simulink model "BoostPFC_Design_HoldUpTest"  (R2024b)
settings: Solver=FixedStepDiscrete  StartTime=0  StopTime=sim_stop_time  FixedStep=Ts_sim  RelTol=1e-3
InitFcn:
  | modelFile=get_param(bdroot,'FileName'); run(fullfile(fileparts(modelFile),'BoostPFC_Design_HoldUp_Init.m')); clear modelFile
values from neighbouring files (symbols this model uses):
  actual_peak_cycle_limit_A = 4.00    (= 4)    [BoostPFC_Design_ControlledStartup_Init.m]
  actual_peak_fault_limit_A = 4.50    (= 4.5)    [BoostPFC_Design_ControlledStartup_Init.m]
  C_out = 2200e-6    (= 0.0022)    [BoostPFC_Design_Init.m]
  duty_max = 0.95    [BoostPFC_Design_Init.m]
  duty_min = 0.0    (= 0)    [BoostPFC_Design_Init.m]
  f_line = 50    [BoostPFC_Design_Init.m]
  f_sw = 50e3    (= 50000)    [BoostPFC_Design_Init.m]
  hold_up_command_time_s = 1.200    (= 1.2)    [BoostPFC_Design_HoldUp_Init.m]
  Ipk_limit = 4.5    [BoostPFC_Design_Init.m]
  Ki_i = Kp_i*2*pi*fz_i    (= 695.807110277)    [BoostPFC_Design_Init.m]
  Ki_v = Kp_v*2*pi*fz_v    [BoostPFC_Design_Init.m]
  Kp_i = 2*pi*fc_i_target*L_boost/Vout_ref    (= 0.221482282078)    [BoostPFC_Design_Init.m]
  Kp_v = 2*pi*fc_v_target/gvi_coefficient    [BoostPFC_Design_Init.m]
  L_boost = 470e-6    (= 0.00047)    [BoostPFC_Design_Init.m]
  load_conductance_ramp_time_s = 80e-3    (= 0.08)    [BoostPFC_Design_LoadConnection_Init.m]
  load_connection_strategy = 0    [BoostPFC_Design_LoadConnection_Init.m]
  load_stage_interval_s = 40e-3    (= 0.04)    [BoostPFC_Design_LoadConnection_Init.m]
  load_step_mode = 0    [BoostPFC_Design_Init.m]    (also in Run_BoostPFC_Design_Cases.m = stepModes(caseIndex))
  load_step_time = 0.45    [BoostPFC_Design_Init.m]    (also in Run_BoostPFC_Design_Cases.m = 0.7)
  precharge_resistance = 10    [BoostPFC_Design_Init.m]
  Rds_on_effective = Rds_on    (= 0.04)    [BoostPFC_Design_Init.m]    (also in Run_Ideal_Component_Comparison.m = 0)
  rL_effective = rL    (= 0.1)    [BoostPFC_Design_Init.m]    (also in Run_Ideal_Component_Comparison.m = 0)
  Rload_nominal = 40    [BoostPFC_Design_Init.m]
  Rload_precharge = 1e9    (= 1000000000)    [BoostPFC_Design_Init.m]
  startup_current_limit_initial_A = 0.50    (= 0.5)    [BoostPFC_Design_ControlledStartup_Init.m]
  startup_ramp_time_s = 100e-3    (= 0.1)    [BoostPFC_Design_ControlledStartup_Init.m]
  Ts_sim = 1 / (20 * f_sw)    (= 1e-06)    [BoostPFC_Design_Init.m]
  Vac_rms = 24    [BoostPFC_Design_Init.m]    (also in Run_BoostPFC_Design_Cases.m)
  Vf_boost_effective = Vf_boost    (= 0.65)    [BoostPFC_Design_Init.m]    (also in Run_Ideal_Component_Comparison.m = 0)
  Vf_bridge_effective = Vf_bridge    (= 0.7)    [BoostPFC_Design_Init.m]    (also in Run_Ideal_Component_Comparison.m = 0)
  Vout_ref = 40    [BoostPFC_Design_Init.m]
settings Model: Creator=86133  LastModifiedBy=86133
settings DataIOCC: SaveOutput=off  SaveTime=off

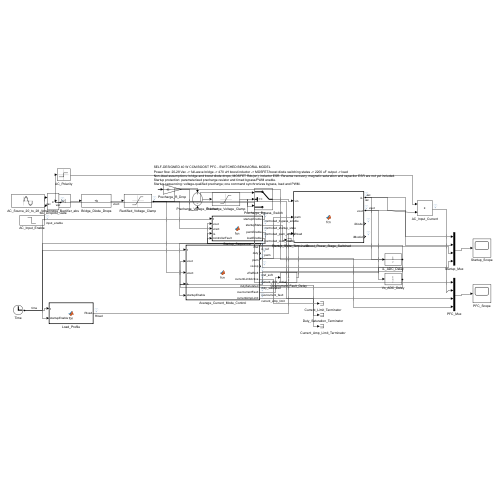
[thumbnail: Simulink's stored preview of the top-level diagram]
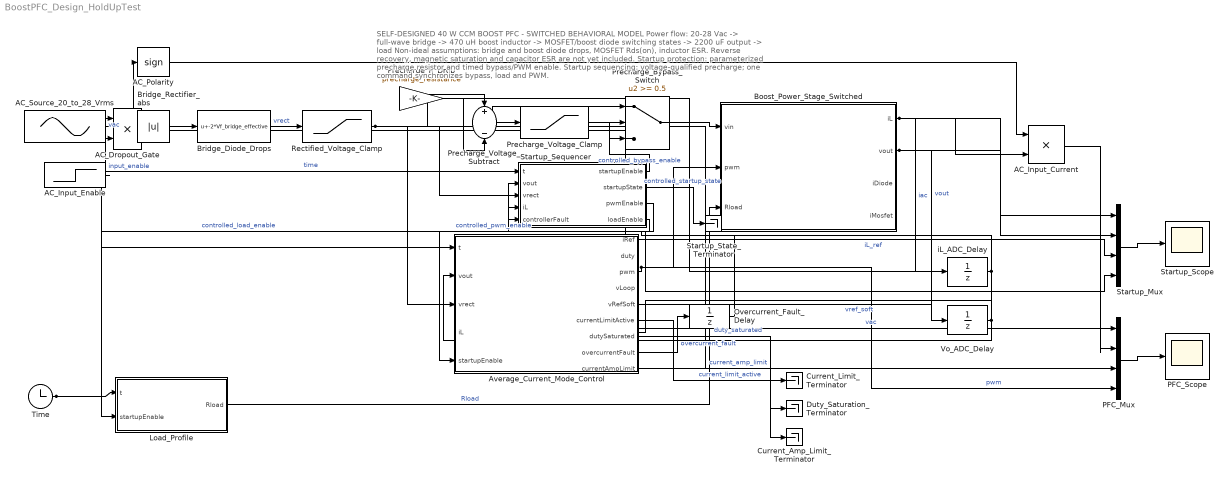
== system BoostPFC_Design_HoldUpTest ==
  note: SELF-DESIGNED 40 W CCM BOOST PFC - SWITCHED BEHAVIORAL MODEL
      | Power flow: 20-28 Vac -> full-wave bridge -> 470 uH boost inductor -> MOSFET/boost diode switching states -> 2200 uF output -> load
      | Non-ideal assumptions: bridge and boost diode drops, MOSFET Rds(on), inductor ESR. Reverse recovery, magnetic saturation and capacitor ESR are not yet included.
      | Startup protection: parameterized precharge resistor and timed bypass/PWM enable.
      | Startup sequencing: voltage-qualified precharge; one command synchronizes bypass, load and PWM.
  AC_Dropout_Gate : Product  Inputs=**
  AC_Input_Current : Product
  AC_Input_Enable : Step  Time=hold_up_command_time_s  Before=1  After=0  SampleTime=Ts_sim
  AC_Polarity : Signum
  AC_Source_20_to_28_Vrms : Sin  Amplitude=sqrt(2)*Vac_rms  Frequency=2*pi*f_line  SampleTime=Ts_sim
  Average_Current_Mode_Control : MATLAB Function  TreatAsAtomicUnit=on
  Boost_Power_Stage_Switched : MATLAB Function  TreatAsAtomicUnit=on
  Bridge_Diode_Drops : Bias  Bias=-2*Vf_bridge_effective  SaturateOnIntegerOverflow=off
  Bridge_Rectifier_abs : Abs  SaturateOnIntegerOverflow=off
  Current_Amp_Limit_Terminator : Terminator
  Current_Limit_Terminator : Terminator
  Duty_Saturation_Terminator : Terminator
  Load_Profile : MATLAB Function  TreatAsAtomicUnit=on
  Overcurrent_Fault_Delay : UnitDelay  SampleTime=Ts_sim  HasFrameUpgradeWarning=on
  PFC_Mux : Mux
  PFC_Scope : Scope
  Precharge_Bypass_Switch : Switch  Threshold=0.5  SaturateOnIntegerOverflow=off  InputSameDT=off
  Precharge_R_Drop : Gain  Gain=precharge_resistance
  Precharge_Voltage_Clamp : Saturate  UpperLimit=inf  LowerLimit=0
  Precharge_Voltage_Subtract : Sum  Inputs=+-
  Rectified_Voltage_Clamp : Saturate  UpperLimit=inf  LowerLimit=0
  Startup_Mux : Mux
  Startup_Scope : Scope
  Startup_Sequencer : MATLAB Function  TreatAsAtomicUnit=on
  Startup_State_Terminator : Terminator
  Time : Clock
  Vo_ADC_Delay : UnitDelay  SampleTime=Ts_sim  HasFrameUpgradeWarning=on
  iL_ADC_Delay : UnitDelay  SampleTime=Ts_sim  HasFrameUpgradeWarning=on
  wires:
  Bridge_Rectifier_abs/1 -> Bridge_Diode_Drops/1
  Bridge_Diode_Drops/1 -> Rectified_Voltage_Clamp/1  "vrect"
  Time/1 -> Load_Profile/1(t), Average_Current_Mode_Control/1(t), Startup_Sequencer/1(t)  "time"
  Rectified_Voltage_Clamp/1 -> Average_Current_Mode_Control/3(vrect), PFC_Mux/3, Precharge_Voltage_Subtract/1, Precharge_Bypass_Switch/1, Startup_Sequencer/3(vrect)
  Average_Current_Mode_Control/3(pwm) -> Boost_Power_Stage_Switched/2(pwm), PFC_Mux/4  "pwm"
  Load_Profile/1(Rload) -> Boost_Power_Stage_Switched/3(Rload)  "Rload"
  Vo_ADC_Delay/1 -> Average_Current_Mode_Control/2(vout), Startup_Sequencer/2(vout)
  iL_ADC_Delay/1 -> Average_Current_Mode_Control/4(iL), Precharge_R_Drop/1, Startup_Sequencer/4(iL)
  Boost_Power_Stage_Switched/1(iL) -> iL_ADC_Delay/1, AC_Input_Current/2, Startup_Mux/2  "iac"
  Boost_Power_Stage_Switched/2(vout) -> Vo_ADC_Delay/1, Startup_Mux/1  "vout"
  AC_Polarity/1 -> AC_Input_Current/1
  Average_Current_Mode_Control/1(iRef) -> Startup_Mux/3  "iL_ref"
  Average_Current_Mode_Control/5(vRefSoft) -> Startup_Mux/4  "vref_soft"
  Startup_Mux/1 -> Startup_Scope/1
  AC_Input_Current/1 -> PFC_Mux/2
  PFC_Mux/1 -> PFC_Scope/1
  Precharge_R_Drop/1 -> Precharge_Voltage_Subtract/2
  Precharge_Voltage_Subtract/1 -> Precharge_Voltage_Clamp/1
  Precharge_Voltage_Clamp/1 -> Precharge_Bypass_Switch/3
  Precharge_Bypass_Switch/1 -> Boost_Power_Stage_Switched/1(vin)
  Startup_Sequencer/1(startupEnable) -> Precharge_Bypass_Switch/2  "controlled_bypass_enable"
  Startup_Sequencer/2(startupState) -> Startup_State_Terminator/1  "controlled_startup_state"
  Startup_Sequencer/3(pwmEnable) -> Average_Current_Mode_Control/5(startupEnable)  "controlled_pwm_enable"
  Startup_Sequencer/4(loadEnable) -> Load_Profile/2(startupEnable)  "controlled_load_enable"
  Average_Current_Mode_Control/8(overcurrentFault) -> Overcurrent_Fault_Delay/1  "overcurrent_fault"
  Overcurrent_Fault_Delay/1 -> Startup_Sequencer/5(controllerFault)
  Average_Current_Mode_Control/6(currentLimitActive) -> Current_Limit_Terminator/1  "current_limit_active"
  Average_Current_Mode_Control/7(dutySaturated) -> Duty_Saturation_Terminator/1  "duty_saturated"
  Average_Current_Mode_Control/9(currentAmpLimit) -> Current_Amp_Limit_Terminator/1  "current_amp_limit"
  AC_Source_20_to_28_Vrms/1 -> AC_Dropout_Gate/1  "vac"
  AC_Input_Enable/1 -> AC_Dropout_Gate/2  "input_enable"
  AC_Dropout_Gate/1 -> Bridge_Rectifier_abs/1, AC_Polarity/1, PFC_Mux/1  "vac"

== matlab function BoostPFC_Design_HoldUpTest/Average_Current_Mode_Control ==
  data: t input double size=1; iRef output double size=1; vout input double size=1; vrect input double size=1; iL input double size=1; duty output double size=1; pwm output double size=1; vLoop output double size=1; vRefSoft output double size=1; startupEnable input double size=1; currentLimitActive output double size=1; dutySaturated output double size=1; overcurrentFault output double size=1; currentAmpLimit output double size=1; Ts_sim parameter double size=1; f_sw parameter double size=1; Vout_ref parameter double size=1; Vac_rms parameter double size=1; Kp_v parameter double size=1; Ki_v parameter double size=1; Kp_i parameter double size=1; Ki_i parameter double size=1; Ipk_limit parameter double size=1; duty_min parameter double size=1; duty_max parameter double size=1; startup_ramp_time_s parameter double size=1; startup_current_limit_initial_A parameter double size=1; actual_peak_cycle_limit_A parameter double size=1; actual_peak_fault_limit_A parameter double size=1
function [iRef,duty,pwm,vLoop,vRefSoft,currentLimitActive,dutySaturated,overcurrentFault,currentAmpLimit] = fcn(t,vout,vrect,iL,startupEnable, Ts_sim, f_sw, Vout_ref, Vac_rms, Kp_v, Ki_v, Kp_i, Ki_i, Ipk_limit, duty_min, duty_max, startup_ramp_time_s, startup_current_limit_initial_A, actual_peak_cycle_limit_A, actual_peak_fault_limit_A)
% Average-current control with reference ramp and measured peak limiter.
persistent intV intI carrier enableTime startVoltage faultLatched
if isempty(intV), intV=0; intI=0; carrier=0; enableTime=-1; startVoltage=0; faultLatched=false; end
if startupEnable>=0.5 && iL>=actual_peak_fault_limit_A, faultLatched=true; end
overcurrentFault=double(faultLatched);
currentLimitActive=0; dutySaturated=0; currentAmpLimit=startup_current_limit_initial_A;
if startupEnable<0.5 || faultLatched
 intV=0; intI=0; carrier=0; enableTime=-1;
 iRef=0; duty=0; pwm=0; vLoop=0; vRefSoft=vout; return;
end
if enableTime<0, enableTime=t; startVoltage=vout; end
alpha=min(max((t-enableTime)/startup_ramp_time_s,0),1);
vRefSoft=startVoltage+(Vout_ref-startVoltage)*alpha;
currentAmpLimit=startup_current_limit_initial_A+alpha*(Ipk_limit-startup_current_limit_initial_A);
eV=vRefSoft-vout; vUnsat=Kp_v*eV+intV;
vLoop=min(max(vUnsat,0),currentAmpLimit);
if (vUnsat==vLoop)||(vUnsat>currentAmpLimit&&eV<0)||(vUnsat<0&&eV>0), intV=intV+Ki_v*Ts_sim*eV; end
vPeak=max(sqrt(2)*Vac_rms,1); iRef=min(currentAmpLimit,max(0,vLoop*vrect/vPeak));
eI=iRef-iL; dFeedforward=1-vrect/max(Vout_ref,1); dUnsat=dFeedforward+Kp_i*eI+intI;
duty=min(max(dUnsat,duty_min),duty_max);
dutySaturated=double(dUnsat<=duty_min || dUnsat>=duty_max);
if (dUnsat==duty)||(dUnsat>duty_max&&eI<0)||(dUnsat<duty_min&&eI>0), intI=intI+Ki_i*Ts_sim*eI; end
carrier=carrier+f_sw*Ts_sim; if carrier>=1, carrier=carrier-floor(carrier); end
if iL>=actual_peak_cycle_limit_A
 currentLimitActive=1; pwm=0;
else
 pwm=double(duty>carrier);
end

== matlab function BoostPFC_Design_HoldUpTest/Load_Profile ==
  data: t input double size=1; Rload output double size=1; startupEnable input double size=1; load_step_mode parameter double size=1; Rload_nominal parameter double size=1; load_step_time parameter double size=1; Rload_precharge parameter double size=1; load_connection_strategy parameter double size=1; load_stage_interval_s parameter double size=1; load_conductance_ramp_time_s parameter double size=1
function Rload = fcn(t,startupEnable,load_step_mode,Rload_nominal,load_step_time,Rload_precharge,load_connection_strategy, load_stage_interval_s, load_conductance_ramp_time_s)
% The sequencer supplies one common load-permission edge for every strategy.
persistent enableTime previousEnable
if isempty(enableTime), enableTime=0; previousEnable=0; end
if startupEnable>=0.5 && previousEnable<0.5, enableTime=t; end
previousEnable=startupEnable;
if startupEnable<0.5
 Rload=Rload_precharge; return;
end
elapsed=max(t-enableTime,0);
if load_connection_strategy==1
 % Three discrete conductance levels: 160, 80 and 40 ohm.
 if elapsed<load_stage_interval_s
  Rload=4*Rload_nominal;
 elseif elapsed<2*load_stage_interval_s
  Rload=2*Rload_nominal;
 else
  Rload=Rload_nominal;
 end
elseif load_connection_strategy==2
 % Linear load-conductance ramp from effectively open circuit to 1/Rnom.
 alpha=min(max(elapsed/load_conductance_ramp_time_s,0),1);
 conductance=(1-alpha)/Rload_precharge+alpha/Rload_nominal;
 Rload=1/max(conductance,1/Rload_precharge);
elseif load_connection_strategy==0
 Rload=Rload_nominal;
elseif load_step_mode==1
 % Retain the old diagnostic modes for traceability; not used in this study.
 if t<load_step_time, Rload=2*Rload_nominal; else, Rload=Rload_nominal; end
elseif load_step_mode==2
 if t<load_step_time, Rload=Rload_nominal; else, Rload=2*Rload_nominal; end
else
 Rload=Rload_nominal;
end

== matlab function BoostPFC_Design_HoldUpTest/Boost_Power_Stage_Switched ==
  data: vin input size=1; iL output size=1; pwm input size=1; Rload input size=1; vout output size=1; iDiode output size=1; iMosfet output size=1; Ts_sim parameter; L_boost parameter; C_out parameter; rL_effective parameter; Rds_on_effective parameter; Vf_boost_effective parameter
function [iL,vout,iDiode,iMosfet] = fcn(vin,pwm,Rload, Ts_sim, L_boost, C_out, rL_effective, Rds_on_effective, Vf_boost_effective)
% Cycle-resolved switched boost equations.
persistent iState vState
if isempty(iState), iState=0; vState=0; end
loadCurrent=vState/max(Rload,1e-6);
if pwm>=0.5
 di=(vin-iState*(rL_effective+Rds_on_effective))/L_boost; dv=-loadCurrent/C_out; iMosfet=iState; iDiode=0;
else
 if (iState>0)||(vin>vState+Vf_boost_effective)
  di=(vin-vState-Vf_boost_effective-iState*rL_effective)/L_boost; iDiode=max(iState,0); dv=(iDiode-loadCurrent)/C_out;
 else
  di=0; iState=0; iDiode=0; dv=-loadCurrent/C_out;
 end
 iMosfet=0;
end
iState=max(iState+Ts_sim*di,0); vState=max(vState+Ts_sim*dv,0); iL=iState; vout=vState;

== matlab function BoostPFC_Design_HoldUpTest/Startup_Sequencer ==
  data: t input double size=1; startupEnable output double size=1; vout input double size=1; startupState output double size=1; vrect input double size=1; iL input double size=1; pwmEnable output double size=1; loadEnable output double size=1; controllerFault input double size=1; Ts_sim parameter double size=1; safe_output_threshold_V parameter double size=1; safe_rectified_threshold_V parameter double size=1; safe_voltage_difference_max_V parameter double size=1; safe_bypass_current_max_A parameter double size=1; safe_condition_hold_time_s parameter double size=1; safe_bypass_timeout_s parameter double size=1; bypass_settle_min_time_s parameter double size=1; pwm_start_current_max_A parameter double size=1; pwm_start_condition_hold_s parameter double size=1; pwm_start_timeout_s parameter double size=1; startup_ramp_time_s parameter double size=1; Vout_ref parameter double size=1; load_connect_voltage_tolerance_V parameter double size=1; load_connect_stable_time_s parameter double size=1; load_connect_timeout_s parameter double size=1
function [startupEnable,startupState,pwmEnable,loadEnable] = fcn(t,vout,vrect,iL,controllerFault, Ts_sim, safe_output_threshold_V, safe_rectified_threshold_V, safe_voltage_difference_max_V, safe_bypass_current_max_A, safe_condition_hold_time_s, safe_bypass_timeout_s, bypass_settle_min_time_s, pwm_start_current_max_A, pwm_start_condition_hold_s, pwm_start_timeout_s, startup_ramp_time_s, Vout_ref, load_connect_voltage_tolerance_V, load_connect_stable_time_s, load_connect_timeout_s)
% States: 0 precharge, 1 bypass wait, 2 PWM ramp, 3 wait load, 4 run.
% Faults: -1 precharge timeout, -2 overcurrent, -3 startup timeout.
persistent state validDuration stateEntryTime stableDuration
if isempty(state), state=0; validDuration=0; stateEntryTime=0; stableDuration=0; end
if controllerFault>=0.5, state=-2; end
if state==0
 voltageDifference=abs(vrect-vout);
 conditions=(vout>=safe_output_threshold_V) && ...
  (vrect>=safe_rectified_threshold_V) && ...
  (voltageDifference<=safe_voltage_difference_max_V) && ...
  (iL<=safe_bypass_current_max_A);
 if conditions, validDuration=validDuration+Ts_sim; else, validDuration=0; end
 if validDuration>=safe_condition_hold_time_s
  state=1; stateEntryTime=t; validDuration=0;
 elseif t>=safe_bypass_timeout_s
  state=-1;
 end
elseif state==1
 conditions=(t-stateEntryTime>=bypass_settle_min_time_s) && (iL<=pwm_start_current_max_A);
 if conditions, validDuration=validDuration+Ts_sim; else, validDuration=0; end
 if validDuration>=pwm_start_condition_hold_s
  state=2; stateEntryTime=t; validDuration=0;
 elseif t>=pwm_start_timeout_s
  state=-3;
 end
elseif state==2
 if t-stateEntryTime>=startup_ramp_time_s, state=3; stateEntryTime=t; stableDuration=0; end
elseif state==3
 if abs(vout-Vout_ref)<=load_connect_voltage_tolerance_V
  stableDuration=stableDuration+Ts_sim;
 else
  stableDuration=0;
 end
 if stableDuration>=load_connect_stable_time_s
  state=4; stateEntryTime=t;
 elseif t>=load_connect_timeout_s
  state=-3;
 end
end
startupEnable=double(state>=1 && state<=4);
pwmEnable=double(state>=2 && state<=4);
loadEnable=double(state==4);
startupState=double(state);
